simulink library "mssSimulink"  (R2024a)
settings: Solver=ode45  StartTime=0.0  StopTime=10.0  RelTol=1e-3
undefined symbols (not defined in the file): ABC, CN_data, CX_data, CY_data, D, G, Hoerner, K_supply, kt2ms, MA, magnitude, MRB, pathlength, RAO_Amp, RAO_Dir, RAO_Freq, RAO_Phase, RAO_Vel, RAO_yaw_back, RAO_yaw_quant, RAO_yaw_quantization_flag, rho_a, slcm, T_supply, table, vessel, vesselABC
libraries: $bdroot x99, simulink x13
(part 1 of 9)
settings Model: Creator=tristan  LastModifiedBy=thor
settings SolverCC: AlgebraicLoopSolver=TrustRegion
settings DataIOCC: LimitDataPoints=on  SaveFormat=Array  SignalLoggingSaveFormat=ModelDataLogs  ReturnWorkspaceOutputs=off
settings OptimizationCC: BlockReduction=off  BooleanDataType=off  ExpressionDepthLimit=2147483647  LifeSpan=inf
settings DebuggingCC: SaveWithParameterizedLinksMsg=none  UnderspecifiedInitializationDetection=Classic  MergeDetectMultiDrivingBlocksExec=none  SignalResolutionControl=TryResolveAllWithWarning  FcnCallInpInsideContextMsg=warning  UnconnectedInputMsg=warning  UnconnectedOutputMsg=warning  UnconnectedLineMsg=warning  StateNameClashWarn=warning  SFUnexpectedBacktrackingDiag=warning  SFNoUnconditionalDefaultTransitionDiag=warning  SFExecutionAtInitializationDiag=none  ArithmeticOperatorsInVariantConditions=warning
settings HardwareCC: ProdBitPerPointer=32  ProdBitPerSizeT=32  ProdBitPerPtrDiffT=32  ProdLargestAtomicFloat=None  ProdIntDivRoundTo=Undefined  ProdEndianess=Unspecified  ProdWordSize=32  ProdHWDeviceType=32-bit Generic  TargetUnknown=on
settings ModelReferenceCC: EnableRefExpFcnMdlSchedulingChecks=on  PropagateSignalLabelsOutOfModel=off
settings SFSimCC: SimUseLocalCustomCode=off  CustomCodeUndefinedFunction=UseInterfaceOnly
settings RTWCC: RTWUseLocalCustomCode=off  GPUComputeCapability=3.5  DLArmComputeVersion=19.05
settings CodeAppCC: StateflowObjectComments=on
settings GRTTargetCC: TargetLangStandard=C89/C90 (ANSI)  CombineOutputUpdateFcns=off  GRTInterface=on
settings ConfigComp: CovMetricSettings=dw  CovSaveCumulativeToWorkspaceVar=on  CovSaveSingleToWorkspaceVar=on  CovExternalEMLEnable=off

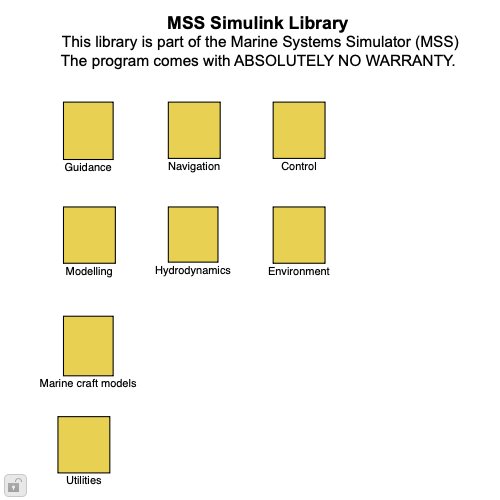
[thumbnail: Simulink's stored preview of the top-level diagram]
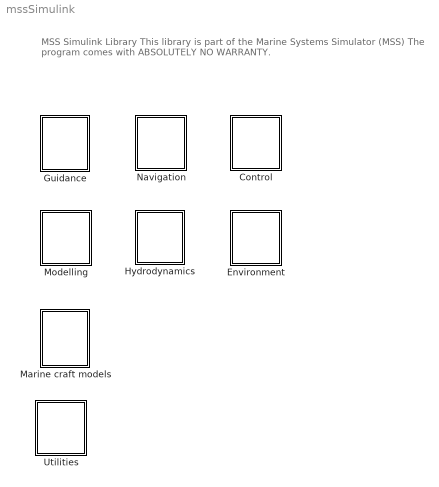
== system mssSimulink ==
  note: MSS Simulink Library
      | This library is part of the Marine Systems Simulator (MSS)
      | The program comes with ABSOLUTELY NO WARRANTY.
  Control : Subsystem
  Environment : Subsystem
  Guidance : Subsystem
  Hydrodynamics : Subsystem
  Marine craft models : Subsystem
  Modelling : Subsystem
  Navigation : Subsystem
  Utilities : Subsystem

== system mssSimulink/Control ==
  Autopilots : Subsystem
  DP : Subsystem

== system mssSimulink/Environment ==
  Current : Subsystem
  Waves : Subsystem
  Wind : Subsystem

== system mssSimulink/Guidance ==
  ALOS guidance law for heading autopilot : MATLAB Function  InitFcn=clear ILOSpsi  TreatAsAtomicUnit=on
  ILOS guidance law for heading autopilot : MATLAB Function  InitFcn=clear ILOSpsi  TreatAsAtomicUnit=on
  LOS guidance law for course autopilot : MATLAB Function  InitFcn=clear LOSchi  TreatAsAtomicUnit=on
  LOS observer : Subsystem  mask(LOS observer){K_f=0.3, alpha=5}
      mask prompts: K_f "Observer gain"; alpha "Bandwidth ratio between the differentiator and the observer, typically 5 to 10"
      mask help:
      | LOSobserver estimates the desired Line-Of-Sight (LOS) angle and rate from a LOS guidance law command, LOScommand[k]. The observer is
      |
      |   LOSangle[k+1] = LOSangle[k] + h * ( LOSrate[k] + K_f * ssa(LOScommand[k] - LOSangle[k]))
      |
      | where the LOS yaw rate is computed using numerical differentiation, LOSrate = T_f*s / (T_f*s + 1) * LOSangle. Exact discretization gives (Fossen 2021, Eqs. B.46-B.47)
      |
      |   LOSratek] = LOSangle[k][k] - xi[k]
      |   xi[k+1] = exp(-h/T_f) * xi[k] + (1 - exp(-h/T_f)) * LOSangle[k]
      |
      | where
      |
      |   K_f: Observer gain, LOSangle (typically 0.1-0.5)
      |   T_f:  Differentiator time constant,  LOSrate = T_f*s / (T_f*s + 1) * LOSangle
      |
      | Typically, the LOSrate loop is chosen 5 times faster than the LOSangle loop, that is 1/T_f = alpha * K_f where alpha = 5
      mask Display:
      | disp('Observer')
      | port_label('output', 2, 'LOSrate')
      | port_label('output', 1, 'LOSangle')
      | port_label('input', 1, 'LOScommand')
  Reference model : Subsystem  mask(3rd-order reference model){v_max=1.0, zeta_d=1.0, w_d=0.1}
      mask prompts: v_max "Max. velocity:"; zeta_d "Relative damping ratio:"; w_d "Natural frequency:"
      mask help: 3rd-order reference model with velocity saturation.
      mask Display:
      | disp('3rd order \nLP-filter')
      | port_label('output', 3, 'acc_d')
      | port_label('output', 2, 'vel_d')
      | port_label('output', 1, 'mag_d')
      | port_label('input', 1, 'ref')
  Waypoint guidance block : Subsystem  mask(Guidance){x_vector=[-800 -500 -200 -50 -200 -250 200 500 500 300 0 -300 -600], y_vector=[100 1800 2000 1500 1000 100 1000 300 -250 -200 100 -600 -1000], method=5th order polynomial, drawmode=off, stop=on, mode=Acc, start=[100 0], final=[0 100], constraint=off}
      mask prompts: x_vector "X value"; y_vector "Y value"; method "Computation method for path generation"; drawmode "Draw an extra plot showing the path with waypoints"; stop "Stop simulation when last waypoint is reached"; mode "Use constraints on acceleration or velocity in the endpoints"; start "Constraints in first waypoint [x, y]. (Only applicable for cubic splines)"; final "Constraints in last waypoint [x, y]. (Only applicable for cubic splines)"; constraint "Use constraints on the derivatives (Only applicable for 5th order)"
      mask help:
      | Way-Point Guidance Block
      | Author:  Jorgen Corneliussen
      | Date:     20 November 2002
      |
      | Creates a three times differentiable path between the waypoints provided. The user can choose between cubic splines and polinomial interpolation.
      |
      | NOTE: You have to supply the actual waypoints for the path generation.
      mask init:
      | if method == 1
      | 	[table, pathlength] = order3(x_vector,y_vector, drawmode, mode, start(1), final(1), start(2), final(2));
      | elseif method == 2
      | 	[table, pathlength] = order5(drawmode, constraint, x_vector, y_vector);
      | else
      | 	disp('Error in block initialization')
      | end
      mask Help:
      | <p>Way-Point Guidance Block<br>
      |   Author: Jorgen Corneliussen<br>
      |   Date: 20 November 2002</p>
      | <ul>
      |   <li> The input vectors must be of the same length, and contain the coordinates
      |     of the waypoints.</li>
      |   <li>If chosen, the block can draw an extra plot showing the path and the waypoints.</li>
      |   <li> The field &quot;Computation method&quot; allows the user to choose between
      |     a third and fifth order polynomal for path generation. </li>
      |   <li>If &quot;Stop simulation&quot; is not checked, the velocity input to the
      |     block is set to zero when the last waypoint is reached. </li>
      |   <li>For the third order algorithm, the user can choose between having endpoint
      |     constraints in velocity or acceleration. The values must be provided in the
      |     specified fields.</li>
      |   <li>For the fifth order polynomial, the user can choose to constrain the derivatives
      |     in the waypoints. This might in some cases reduce oscillations.<br>
      |   </li>
      | </ul>
      mask TypeOptions method: Cubic spline | 5th order polynomial
      mask TypeOptions mode: Vel | Acc
      mask Display:
      | image(imread('simulink/figs/compass.jpg'))
      | 
      | color('black'); port_label('output', 1, 'xy')
      | color('black'); port_label('output', 2, 'eta_vec')
      | color('black'); port_label('output', 3, 'vs_tot')
      | 
      | color('black'); port_label('input', 1, 'ud_total')
      | color('black'); port_label('input', 2, 'theta')
  "Zigzag test rudder command " : Subsystem  mask(Z- Manoeuvre test or Zig-Zag test){RL=[]}
      mask prompts: RL "Maximum rudder angle [rad]:"
      mask help:
      | This block generates the rudder command for a Z-manoeuvre test
      | IMO A601, ITTC 1975, SNAME 1989.
      | Copyright (C) 2005 NTNU
      |  Author: Tristan Perez

== system mssSimulink/Hydrodynamics ==
  6-DOF DP model (zero-speed model with fluid memory) : Subsystem  mask(6 DOF zero speed model){ABC=vesselABC, rho=1025, Axc=0.9*vessel.main.T*vessel.main.B, Ayc=0.9*vessel.main.T*vessel.main.Lpp, CX=1, CY_2D=Hoerner(vessel.main.B,vessel.main.T)}
      mask prompts: ABC "Structure containing model parameters and the fluid memory effects"; rho "Density of water (kg/m3)"; Axc "Frontal projected current area Axc (m2)"; Ayc "Laterall projected current area Ayc (m2)"; CX "Current (drag) coefficient in surge CX"; CY_2D "2D drag coefficient in sway CY_2D"
      mask help: System block containing the zero speed 6 DOF equations of motion including fluid memory effetcs.
  6-DOF maneuvering model (unified model with fluid memory) : Subsystem  mask(ShipX (Veres) 6 DOF unified DP and maneuvering model){ABC=vesselABC, rho=1025, Axc=0.9*vessel.main.T*vessel.main.B, Ayc=0.9*vessel.main.T*vessel.main.Lpp, CX=1, CY_2D=Hoerner(vessel.main.B,vessel.main.T)}
      mask prompts: ABC "Structure containing the fluid memory effects"; rho "Density of water (kg/m3)"; Axc "Frontal projected current area (m2)"; Ayc "Lateral projected current area (m2)"; CX "Current (drag) coefficient in surge CX"; CY_2D "2D drag coefficient in sway CY_2D"
      mask help:
      | System block containing the Shipx (Veres) 6 DOF unified DP and maneuvering model. The  6 DOF equations of motion also includes fluid memory effetcs. The data structure:
      |
      |    ABC.*           (>> load ABC )
      |
      | is generated using the Matlab script:
      |
      |    >> veres2ABC.m
      |
      | This script computes the retardation functions using state-space model approximations. It is also possible to include frequency-dependent viscous effects my editing the script.
      |
      | Author: Thor I. Fossen
      | -------------------------------------------------------------------------------------------------------------------------------------------------------
      | Reference:
      | T. I. Fossen and Ø. Smogeli (2004). Nonlinear Time-Domain Strip Theory Formulation for Low-Speed Maneuvering and Station-Keeping, Modelling, Identification and Control, MIC-25 (4):201-221.
      |
      | T. I. Fossen. A Nonlinear Unified State-Space Model for Ship Maneuvering and Control in a Seaway.  Journal of Bifurcation and Chaos (ENOC'05 Plenary), 2005.
  Cross-flow drag and surge resistance : Subsystem  TreatAsAtomicUnit=on  mask(Cross-flow drag and surge resistance){N=20, Lpp=vessel.main.Lpp, CD=0.5, Cx=0.5, Ax=100, Ay=500, rho_w=1025}
      mask prompts: N "Number of cross sections"; Lpp "Length between perpendiculars (m)"; CD "2D transversal drag coefficient CY  (-)"; Cx "3D drag coefficient in surge (-)"; Ax "Frontal current area Ax (m2)"; Ay "Transversal area (m2)"; rho_w "Density of water (kg/m^3)"
      mask help:
      | The viscous current loads in sway and yaw are computed using the cross-flow principle (pp. 187-197, Faltinsen 1990). 2-D drag coefficients CY_2D are used for each section of the hull. Integration over the length Lpp of the ship is performed using the trapezoidal rule. The forces are:
      |
      | Y = 0.5*rho_w*(Ay/Lpp)*CY_2D*Integral_{-0.5*Lpp}^{0.5*Lpp}  (v+x*r)|v+x*r| dx
      | N = 0.5*rho_w*(Ay/Lpp)*CY_2D*Integral_{-0.5*Lpp}^{0.5*Lpp}  x*(v+x*r)|v+x*r| dx
      |
      | where CY_2D is the 2D drag coefficient e.g. computed using Hoerner's formula.
      |
      | In surge the viscous resistance is modelled as quadratic drag:
      |
      | X = 0.5*rho_w*CX*Ax*u*|u|
      |
      | where Cx is the 3D drag coefficient in surge.
      |
      | Author: Thor I. Fossen
      mask init:
      | % ITTC drag
      | epsilon = 201; % ensure that log10(Rn)>2.0
      | 
      | Rn_min = 1e6;  % minimum Reynold's tall
      | %Ct_max = 0.075*(1+k)/(log10(Rn_min)-2)^2;
      | 
      | %S = Lpp*(B+2*T);
      mask Help:
      | <p>The viscous current loads in sway and yaw are computed using the cross-flow principle (pp. 187-197, Faltinsen 1990). 2-D drag coefficients CY_2D are used for each section of the hull. Integration over the length L of the ship is performed using the trapezoidal rule. The forces are:</p>
      | <p>Y = 0.5*rho_w*(Ay/Lpp)*CY_2D*Integral_{-0.5*Lpp}^{0.5*Lpp}  (v+x*r)|v+x*r| dx</p>
      | <p>N = 0.5*rho_w*(Ay/Lpp)*CY_2D*Integral_{-0.5*Lpp}^{0.5*Lpp}  x*(v+x*r)|v+x*r| dx</p>
      | where CY_2D is the 2D drag coefficient e.g. computed using Hoerner's formula.
      | <p>
      | In surge the viscous resistance is modelled as quadratic drag:
      | </p>
      | <p>
      | X = 0.5*rho_w*CX*Ax*u*|u|
      | </p>
      | <p>where Cx is the 3D drag coefficient in surge.<br>
      | </p>
      | <p>Author: Thor I. Fossen</p>
  Fluid memory effetcs : Subsystem
  Motion RAO (U=0) : Subsystem  mask(Motion RAO){RAO_Freq=vessel.motionRAO.w, RAO_Dir=vessel.headings, RAO_Vel=vessel.velocities, RAO_Amp=vessel.motionRAO.amp, RAO_Phase=vessel.motionRAO.phase, RAO_add_omega_0=on, RAO_add_omega_inf=on, RAO_yaw_quantization_flag=on, RAO_yaw_quant=5*pi/180, RAO_yaw_back=1.2*pi/180, RAO_speed_backlash_flag=on, RAO_speed_back=2, RAO_smoothing_flag=on}
      mask prompts: RAO_Freq "Vector of frequencies RAO_Freq (rad/s)"; RAO_Dir "Vector of directions RAO_Dir (rad)"; RAO_Vel "Vector of velocities RAO_Vel (m/s)"; RAO_Amp "6DOF Cell array with tables of Amplitudes RAO_Amp"; RAO_Phase "6DOF Cell array with tables of Phases RAO_Phase (rad)"; RAO_add_omega_0 "Add asymptotic RAO values for omega = 0"; RAO_add_omega_inf "Add asymptotic RAO values for omega = inf"; RAO_yaw_quantization_flag "LF estimator for yaw angle table lookup (backlash and quantization)"; RAO_yaw_quant "LF yaw angle quantization interval [rad]"; RAO_yaw_back "LF yaw angle backlash width [rad] (typically 1/4 of the quantization interval)"; RAO_speed_backlash_flag "Speed lookup backlash (avoid rapid speed data switching)"; RAO_speed_back "Speed backlash widht [m/s]"; RAO_smoothing_flag "Smooth the output to avoid switching transients due to table lookup"
      mask help:
      | Calculate the wave-frequency motion of a vessel in 6 degrees-of-freedom (DOF) from its Motion Response Amplitude Operators (Motion RAOs) and a sea state defined by a set of harmonic waves. The block takes the "Waves" bus from the MSS Waves block as input, as well as the vessel low-frequency (LF) motion in terms of the generalized position vector eta_LF and mean surge velocity U. See help for details.
      |
      | Copyright (C) NTNU 2005
      | Author: Oyvind N. Smogeli, 2005-05-03
      mask init:
      | % use only nonzero increasing velocities, if zero element add eps
      | Nvel = length(RAO_Vel);
      | 
      | if Nvel == 1
      |     RAO_Vel = [0 1e10];   % use one data set for U=0 and one dummy set for u=1e10
      |     Nvel = 2;
      | end
      | 
      | for dof = 1:6
      |     TempA{dof}  = RAO_Amp{dof}(:,:,1:Nvel);
      |     TempP{dof}  = RAO_Phase{dof}(:,:,1:Nvel);
      | end
      | 
      | clear RAO_Amp RAO_Phase
      | 
      | RAO_Amp   = TempA;
      | RAO_Phase = TempP;
      | 
      | % Add RAO values for zero frequency: use values for lowest given frequency
      | if RAO_add_omega_0 > 0
      | 	
      | 	if min(RAO_Freq) > 0
      | 				
      | 		RAO_Freq = [0 RAO_Freq];
      | 		
      | 		for dofno = 1:6
      | 			RAO_Amp{dofno} = [RAO_Amp{dofno}(1,:,:); RAO_Amp{dofno}];
      | 			RAO_Phase{dofno} = [RAO_Phase{dofno}(1,:,:); RAO_Phase{dofno}];
      | 		end
      | 	
      | 	end
      | 	
      | end
      | 
      | % Add RAO values for high frequency: use values for highest given frequency
      | maxfreq = 10;
      | if RAO_add_omega_inf > 0
      | 
      | 	if max(RAO_Freq) < maxfreq
      | 			
      | 		newfreq = 2*max(RAO_Freq) - RAO_Freq(length(RAO_Freq)-1);
      |         if newfreq > maxfreq
      |             newfreq = maxfreq - 0.1;
      |         end
      | 		
      | 		RAO_Freq = [RAO_Freq newfreq maxfreq];
      | 		
      | 		for dofno = 1:6
      | 			RAO_Amp{dofno} = [RAO_Amp{dofno} ; zeros(2, length(RAO_Dir), length(RAO_Vel))];
      | 			RAO_Phase{dofno} = [RAO_Phase{dofno} ; zeros(2, length(RAO_Dir), length(RAO_Vel))];
      | 		end
      | 		
      | 	end
      | 
      | end
      mask Help:
      | <b>Part of the Marine Systems Simulator: MSS</b><br>
      | <br>
      | Calculate the wave-frequency motion of a vessel in 6 degrees-of-freedom (DOF)
      | from its Motion Response Amplitude Operators (Motion RAOs) and a sea state
      | defined by a set of harmonic waves. The block takes the &quot;Waves&quot; bus from the MSS
      | Waves block as input, as well as the vessel low-frequency (LF) motion in terms
      | of the generalized position vector Eta_LF and surge velocity U.<p>
      | The Motion RAOs are defined in terms of a vector of frequencies (RAO_Freq), a
      | vector of directions (RAO_Dir), a vector of velocities (RAO_Dir), a 6DOF cell
      | array of 3D matrices with amplitudes (RAO_Amp), and a 6DOF cell array of 3D
      | matrices with phases (RAO_Phase), which are all input in the block mask. The
      | first dimension of the 3D matrices corresponds to the frequencies, the second to
      | the directions, and the third to the velocities, such that e.g. the amplitude
      | amp in heave (DOF #3) for frequency number n_f, direction number n_d and
      | velocity number n_v can be found from a = RAO_Amp{3}(n_f, n_d, n_v). </p>
      | <p><b>Inputs:</b></p>
      | <p>Waves:&nbsp;&nbsp;&nbsp;&nbsp;&nbsp;&nbsp;&nbsp;&nbsp;&nbsp;&nbsp;&nbsp; Bus
      | containing the following signals<br>
      | &nbsp;&nbsp;&nbsp; Zeta_a:&nbsp;&nbsp;&nbsp;&nbsp;&nbsp;&nbsp;&nbsp; Vector of harmonic wave amplitudes [m]<br>
      | &nbsp;&nbsp;&nbsp; Omega:&nbsp;&nbsp;&nbsp;&nbsp;&nbsp;&nbsp; Vector of harmonic wave frequencies [rad/s]<br>
      | &nbsp;&nbsp;&nbsp; Phase:&nbsp;&nbsp;&nbsp;&nbsp;&nbsp;&nbsp;&nbsp;&nbsp; Vector of harmonic wave phases (random) [rad]<br>
      | &nbsp;&nbsp;&nbsp; Wavenum:&nbsp;&nbsp;&nbsp; Vector of harmonic wave numbers [1/m]<br>
      | &nbsp;&nbsp;&nbsp; Psi:&nbsp;&nbsp;&nbsp;&nbsp;&nbsp;&nbsp;&nbsp;&nbsp;&nbsp;&nbsp;&nbsp;&nbsp;&nbsp; Vector of harmonic wave directions [rad]</p>
      | <p>eta_LF:&nbsp;&nbsp;&nbsp;&nbsp;&nbsp;&nbsp;&nbsp;&nbsp;&nbsp;&nbsp;&nbsp;
      | Generalized 6DOF n-frame low-frequency position vector [x (m), y (m), z (m),
      | theta (rad), phi (rad), psi (rad)]<br>
      | U:&nbsp;&nbsp;&nbsp;&nbsp;&nbsp;&nbsp;&nbsp;&nbsp;&nbsp;&nbsp;&nbsp;&nbsp;&nbsp;&nbsp;&nbsp;&nbsp;&nbsp;&nbsp;&nbsp;
      | Low-frequency (mean) surge velocity&nbsp; [m/s]</p>
      | <p><b>Outputs:</b></p>
      | <p>eta_WF:&nbsp;&nbsp;&nbsp;&nbsp;&nbsp;&nbsp;&nbsp;&nbsp;&nbsp; Generalized
      | 6DOF n-frame wave-frequency position vector [x (m), y (m), z (m), theta (rad),
      | phi (rad), psi (rad)]<br>
      | nu_WF:&nbsp;&nbsp;&nbsp;&nbsp;&nbsp;&nbsp;&nbsp;&nbsp;&nbsp;&nbsp; Generalized
      | 6DOF h-frame wave-frequency velocity vector [u (m/s), v (m/s), w (m/s), p
      | (rad/s), q (rad/s), r (rad/s)]<br>
      | nu_dot_WF:&nbsp;&nbsp;&nbsp;&nbsp; Generalized 6DOF h-frame wave-frequency
      | acceleration vector d/dt([u (m/s), v (m/s), w (m/s), p (rad/s), q (rad/s), r
      | (rad/s)])</p>
      | <p><b>Model validity:</b></p>
      | <p>The validity of the block is dependent on the validity of the given
      | RAO data set.</p>
      | <p>A proper RAO to be used with this block should contain at least 1 velocity, 5
      | directions (e.g. 0, 45, 90, 135 and 180 degrees) and 10-20 frequencies, for all
      | 6 DOF (surge, sway, heave, roll, pitch, yaw).</p>
      | <p>The block performs linear interpolation in frequencies and directions, and
      | uses the data set for the velocity closest to the input velocity (i.e. 'nearest'
      | interpolation in velocity). If the block recieves an input wave frequency or relative
      | wave direction outside the span of the data vectors RAO_Freq or RAO_Dir
      | respectively, the simulation stops and an error is returned. This means that a well-defined
      | RAO must contain data for both 0 and 180 degrees, and for frequencies covering
      | the desired range of wave frequencies. If desired, asymptotic values can be
      | automatically added for zero and infinity frequency to avoid runtime errors if
      | the wave freqeuncy exceeds the values in RAO_Freq (see checkboxes in the mask). </p>
      | <p>IMPORTANT NOTE: The RAO theory upon which this block is based is in reality
      | only valid when the vessel low-frequency (h-frame) motion is a constant surge
      | velocity only, and the vessel is performing wave-frequency oscillations about
      | the steadily translating h-frame.This means that the outputs from the block when
      | manoeuvering -- i.e. changing the surge velocity and/or yaw angle -- must be
      | interpreted with some care. A jump in the output must be expected when changing
      | between two velocity data sets, and frequency warping expected when changing the
      | yaw angle (due to interpolation in the phase). It is therefore recommended to
      | use backlash on the input velocity to avoid transient switching, and a quantized
      | yaw angle with backlash. The latter will lead to jump in the ouput when the yaw
      | angle changes from one quantizied value to another, but will give better results
      | when keeping within one quantizer interval. The quantized yaw angle with
      | backlash and velocity with backlash are available as options via checkboxes in
      | the mask. If either of these are activated, proper values for the yaw
      | quantization interval, yaw backlash width, and the the speed backlash width
      | respectively must be set. Typical values could be a yaw quantization interval of
      | 5 degrees, yaw backlash width of 1/4-1/5 of the quantization interval, and speed
      | backlash width of 1 m/s. To avoid the most rapid transients when switching
      | between data sets, output smoothing is available as an option in the mask. If
      | this is enabled, the output during a transent is rate limited according to the
      | fastest recorded signal rate during normal operation.</p>
      | <p><b>Example mask input:</b></p><p>
      | As an example, the format of the mask input for 2 velocities, 3 directions and 5
      | frequencies is as follows:<p>RAO_Freq = [f1 f2 f3 f4 f5]<br>
      | RAO_Dir = [d1 d2 d3]<br>
      | RAO_Vel = [v1 v2]<p>Surge:<br>
      | RAO_Amp{1}(:,:,1)&nbsp; = [a1_111 a1_121 a1_131; a1_211 a1_221 a1_231; a1_311
      | a1_321 a1_331; a1_411 a1_421 a1_431; a1_511 a1_521 a1_531]<br>
      | RAO_Amp{1}(:,:,2)&nbsp; = [a1_112 a1_122 a1_132; a1_212 a1_222 a1_232; a1_312
      | a1_322 a1_332; a1_412 a1_422 a1_432; a1_512 a1_522 a1_532]<br>
      | RAO_Phase{1}(:,:,1) = [p1_111 p1_121 p1_131; p1_211 p1_221 p1_231; p1_311 p1_321
      | p1_331; p1_411 p1_421 p1_431; p1_511 p1_521 p1_531]<br>
      | RAO_Phase{1}(:,:,2) = [p1_112 p1_122 p1_132; p1_212 p1_222 p1_232; p1_312 p1_322
      | p1_332; p1_412 p1_422 p1_432; p1_512 p1_522 p1_532]<p>Sway:<br>
      | RAO_Amp{2}(:,:,1)&nbsp; = [a2_111 a2_121 a2_131; a2_211 a2_221 a2_231; a2_311
      | a2_321 a2_331; a2_411 a2_421 a2_431; a2_511 a2_521 a2_531]<br>
      | RAO_Amp{2}(:,:,2)&nbsp; = [a2_112 a2_122 a2_132; a2_212 a2_222 a2_232; a2_312
      | a2_322 a2_332; a2_412 a2_422 a2_432; a2_512 a2_522 a2_532]<br>
      | RAO_Phase{2}(:,:,1) = [p2_111 p2_121 p2_131; p2_211 p2_221 p2_231; p2_311 p2_321
      | p2_331; p2_411 p2_421 p2_431; p2_511 p2_521 p2_531]<br>
      | RAO_Phase{2}(:,:,2) = [p2_112 p2_122 p2_132; p2_212 p2_222 p2_232; p2_312 p2_322
      | p2_332; p2_412 p2_422 p2_432; p2_512 p2_522 p2_532]<p>....<p>Yaw:<br>
      | RAO_Amp{6}(:,:,1)&nbsp; = [a6_111 a6_121 a6_131; a6_211 a6_221 a6_231; a6_311
      | a6_321 a6_331; a6_411 a6_421 a6_431; a6_511 a6_521 a6_531]<br>
      | RAO_Amp{6}(:,:,2)&nbsp; = [a6_112 a6_122 a6_132; a6_212 a6_222 a6_232; a6_312
      | a6_322 a6_332; a6_412 a6_422 a6_432; a6_512 a6_522 a6_532]<br>
      | RAO_Phase{6}(:,:,1) = [p6_111 p6_121 p6_131; p6_211 p6_221 p6_231; p6_311 p6_321
      | p6_331; p6_411 p6_421 p6_431; p6_511 p6_521 p6_531]<br>
      | RAO_Phase{6}(:,:,2) = [p6_112 p6_122 p6_132; p6_212 p6_222 p6_232; p6_312 p6_322
      | p6_332; p6_412 p6_422 p6_432; p6_512 p6_522 p6_532]<p>where now for example the
      | amplitude and phase in sway (DOF 2) for frequency f5, direction d3 and velocity
      | v1 are given by RAO_Amp{2}(5,3,1) = a2_531 and RAO_Phase{2}(5,3,1) = p2_531.<p>
      | <b>Copyright (C) NTNU 2005</b></p>
      | <p><b>Author:</b> Oyvind N. Smogeli, 2005-05-03</p></body>
  WD for heading1 : Subsystem  mask(Force RAO){ForceRAO_Freq=vessel.forceRAO.w, WD_Freq=vessel.driftfrc.w, RAO_Vel=vessel.velocities, ForceRAO_Amp=vessel.forceRAO.amp, ForceRAO_Phase=vessel.forceRAO.phase, WD_Amp=vessel.driftfrc.amp, RAO_add_omega_0=on, RAO_add_omega_inf=on}
      mask prompts: ForceRAO_Freq "Vector of frequencies ForceRAO_Freq (rad/s)"; WD_Freq "Vector of frequencies WD_Freq (rad/s)"; RAO_Vel "Vector of velocities RAO_Vel (m/s)"; ForceRAO_Amp "6DOF Cell array with tables of Amplitudes ForceRAO_Amp"; ForceRAO_Phase "6DOF Cell array with tables of Phases ForceRAO_Phase (rad)"; WD_Amp "6DOF Cell array with tables of Amplitudes WD_Amp"; RAO_add_omega_0 "Add asymptotic RAO values for omega = 0"; RAO_add_omega_inf "Add asymptotic RAO values for omega = inf"
      mask help:
      | Calculate the 6 degrees-of-freedom (DOF) wave-frequency excitation forces tau_WF for a vessel from its Force Response Amplitude Operators (Force RAOs) and a sea state defined by a set of harmonic waves. The block takes the "Waves" bus from the MSS Waves block as input, as well as the vessel low-frequency (LF) motion in terms of the generalized position vector eta and mean surge velocity U. See help for details.
      |
      | Authors: Oyvind N. Smogeli and Thor I. Fossen, 2005-05-03
      mask init:
      | % use only nonzero increasing velocities, if zero element add eps
      | Nvel = length(RAO_Vel);
      | 
      | if Nvel == 1
      |     RAO_Vel = [0 1e10];   % use one data set for U=0 and one dummy set for u=1e10
      |     Nvel = 2;
      | end
      | 
      | for dof = 1:3
      |     TempWA{dof}  = WD_Amp{dof}(:,:,1:Nvel);
      | end
      | 
      | clear WD_Amp WD_Phase
      | 
      | WD_Amp         = TempWA;
      | 
      | % Add RAO values for zero frequency: use values for lowest given frequency
      | if RAO_add_omega_0 > 0
      | 	 
      | 	if min(WD_Freq) > 0
      |         
      | 		WD_Freq = [0 WD_Freq];
      | 		for dofno = 1:3
      | 			WD_Amp{dofno} = [WD_Amp{dofno}(1,:,:); WD_Amp{dofno}];
      | 		end        
      |         
      | 	end
      | 	
      | end
      | 
      | % Add RAO values for high frequency: use values for highest given frequency
      | maxfreq = 10;
      | if RAO_add_omega_inf > 0
      | 
      | 	if max(WD_Freq) < maxfreq
      | 			
      | 		newfreq = max(WD_Freq) + 0.5*(maxfreq-max(WD_Freq));
      |         
      | 		WD_Freq = [WD_Freq newfreq maxfreq];
      | 		for dofno = 1:3
      | 			WD_Amp{dofno} = [WD_Amp{dofno}; zeros(2, 36, Nvel)];
      | 		end
      | 		
      |     end
      |     
      | end
      mask Help:
      | <b>Part of the Marine Systems Simulator: MSS</b><br>
      | <br>
      | Calculate the 6 degrees-of-freedom (DOF) wave-frequency excitation forces tau_WF
      | for a vessel from its Force Response Amplitude Operators (Force RAOs) and a sea
      | state defined by a set of harmonic waves. The block takes the &quot;Waves&quot; bus from
      | the MSS Waves block as input, as well as the vessel low-frequency (LF) motion in
      | terms of the generalized position vector eta and mean surge velocity U.<p>The Force RAOs are defined in terms of a
      | vector of frequencies (RAO_Freq), a vector of directions (RAO_Dir), a vector of
      | velocities (RAO_Dir), a 6DOF cell array of 3D matrices with amplitudes
      | (RAO_Amp), and a 6DOF cell array of 3D matrices with phases (RAO_Phase), which
      | are all input in the block mask. The first dimension of the 3D matrices
      | corresponds to the frequencies, the second to the directions, and the third to
      | the velocities, such that e.g. the amplitude amp in heave (DOF #3) for frequency
      | number n_f, direction number n_d and velocity number n_v can be found from a =
      | RAO_Amp{3}(n_f, n_d, n_v).</p>
      | <p><b>Inputs:</b></p>
      | <p>Waves:&nbsp;&nbsp;&nbsp;&nbsp;&nbsp;&nbsp;&nbsp;&nbsp;&nbsp;&nbsp;&nbsp; Bus
      | containing the following signals<br>
      | &nbsp;&nbsp;&nbsp; Zeta_a:&nbsp;&nbsp;&nbsp;&nbsp;&nbsp;&nbsp;&nbsp; Vector of harmonic wave amplitudes [m]<br>
      | &nbsp;&nbsp;&nbsp; Omega:&nbsp;&nbsp;&nbsp;&nbsp;&nbsp;&nbsp; Vector of harmonic wave frequencies [rad/s]<br>
      | &nbsp;&nbsp;&nbsp; Phase:&nbsp;&nbsp;&nbsp;&nbsp;&nbsp;&nbsp;&nbsp;&nbsp; Vector of harmonic wave phases (random) [rad]<br>
      | &nbsp;&nbsp;&nbsp; Wavenum:&nbsp;&nbsp;&nbsp; Vector of harmonic wave numbers [1/m]<br>
      | &nbsp;&nbsp;&nbsp; Psi:&nbsp;&nbsp;&nbsp;&nbsp;&nbsp;&nbsp;&nbsp;&nbsp;&nbsp;&nbsp;&nbsp;&nbsp;&nbsp; Vector of harmonic wave directions [rad]</p>
      | <p>eta_LF:&nbsp;&nbsp;&nbsp;&nbsp;&nbsp;&nbsp;&nbsp;&nbsp;&nbsp;&nbsp;&nbsp;
      | Generalized 6DOF n-frame low-frequency position vector [x (m), y (m), z (m),
      | theta (rad), phi (rad), psi (rad)]<br>
      | U:&nbsp;&nbsp;&nbsp;&nbsp;&nbsp;&nbsp;&nbsp;&nbsp;&nbsp;&nbsp;&nbsp;&nbsp;&nbsp;&nbsp;&nbsp;&nbsp;&nbsp;&nbsp;&nbsp;
      | Low-frequency (mean) surge velocity&nbsp; [m/s]</p>
      | <p><b>Outputs:</b></p>
      | <p>tau_WF:&nbsp;&nbsp;&nbsp;&nbsp;&nbsp;&nbsp;&nbsp;&nbsp;&nbsp; Generalized
      | 6DOF h-frame force vector [X (N), Y (N), Z (N), K (Nm), M (Nm), N (Nm)]</p>
      | <p><b>Model validity:</b></p>
      | <p>The validity of the block is dependent on the validity of the given
      | RAO data set.</p>
      | <p>A proper RAO to be used with this block should contain at least 1 velocity, 5
      | directions (e.g. 0, 45, 90, 135 and 180 degrees) and 10-20 frequencies, for all
      | 6 DOF (surge, sway, heave, roll, pitch, yaw).</p>
      | <p>The block performs linear interpolation in frequencies and directions, and
      | uses the data set for the velocity closest to the input velocity (i.e. 'nearest'
      | interpolation in velocity). If the block recieves an input wave frequency or relative
      | wave direction outside the span of the data vectors RAO_Freq or RAO_Dir
      | respectively, the simulation stops and an error is returned. This means that a well-defined
      | RAO must contain data for both 0 and 180 degrees, and for frequencies covering
      | the desired range of wave frequencies. If desired, asymptotic values can be
      | automatically added for zero and infinity frequency to avoid runtime errors if
      | the wave freqeuncy exceeds the values in RAO_Freq (see checkboxes in the mask). </p>
      | <p>IMPORTANT NOTE: The RAO theory upon which this block is based is in reality
      | only valid when the vessel low-frequency (h-frame) motion is a constant surge
      | velocity only, and the vessel is performing wave-frequency oscillations about
      | the steadily translating h-frame.This means that the outputs from the block when
      | manoeuvering -- i.e. changing the surge velocity and/or yaw angle -- must be
      | interpreted with some care. A jump in the output must be expected when changing
      | between two velocity data sets, and frequency warping expected when changing the
      | yaw angle (due to interpolation in the phase). It is therefore recommended to
      | use backlash on the input velocity to avoid transient switching, and a quantized
      | yaw angle with backlash. The latter will lead to jump in the ouput when the yaw
      | angle changes from one quantized value to another, but will give better results
      | when keeping within one quantizer interval. The quantized yaw angle with
      | backlash and velocity with backlash are available as options via checkboxes in
      | the mask. If either of these are activated, proper values for the yaw
      | quantization interval, yaw backlash width, and the the speed backlash width
      | respectively must be set. Typical values could be a yaw quantization interval of
      | 5 degrees, yaw backlash width of 1/4-1/5 of the quantization interval, and speed
      | backlash width of 1 m/s. To avoid the most rapid transients when switching
      | between data sets, output smoothing is available as an option in the mask. If
      | this is enabled, the output during a transent is rate limited according to the
      | fastest recorded signal rate during normal operation.</p>
      | <p><b>Example mask input:</b></p><p>
      | As an example, the format of the mask input for 2 velocities, 3 directions and 5
      | frequencies is as follows:<p>RAO_Freq = [f1 f2 f3 f4 f5]<br>
      | RAO_Dir = [d1 d2 d3]<br>
      | RAO_Vel = [v1 v2]<p>Surge:<br>
      | RAO_Amp{1}(:,:,1)&nbsp; = [a1_111 a1_121 a1_131; a1_211 a1_221 a1_231; a1_311
      | a1_321 a1_331; a1_411 a1_421 a1_431; a1_511 a1_521 a1_531]<br>
      | RAO_Amp{1}(:,:,2)&nbsp; = [a1_112 a1_122 a1_132; a1_212 a1_222 a1_232; a1_312
      | a1_322 a1_332; a1_412 a1_422 a1_432; a1_512 a1_522 a1_532]<br>
      | RAO_Phase{1}(:,:,1) = [p1_111 p1_121 p1_131; p1_211 p1_221 p1_231; p1_311 p1_321
      | p1_331; p1_411 p1_421 p1_431; p1_511 p1_521 p1_531]<br>
      | RAO_Phase{1}(:,:,2) = [p1_112 p1_122 p1_132; p1_212 p1_222 p1_232; p1_312 p1_322
      | p1_332; p1_412 p1_422 p1_432; p1_512 p1_522 p1_532]<p>Sway:<br>
      | RAO_Amp{2}(:,:,1)&nbsp; = [a2_111 a2_121 a2_131; a2_211 a2_221 a2_231; a2_311
      | a2_321 a2_331; a2_411 a2_421 a2_431; a2_511 a2_521 a2_531]<br>
      | RAO_Amp{2}(:,:,2)&nbsp; = [a2_112 a2_122 a2_132; a2_212 a2_222 a2_232; a2_312
      | a2_322 a2_332; a2_412 a2_422 a2_432; a2_512 a2_522 a2_532]<br>
      | RAO_Phase{2}(:,:,1) = [p2_111 p2_121 p2_131; p2_211 p2_221 p2_231; p2_311 p2_321
      | p2_331; p2_411 p2_421 p2_431; p2_511 p2_521 p2_531]<br>
      | RAO_Phase{2}(:,:,2) = [p2_112 p2_122 p2_132; p2_212 p2_222 p2_232; p2_312 p2_322
      | p2_332; p2_412 p2_422 p2_432; p2_512 p2_522 p2_532]<p>...<p>Yaw:<br>
      | RAO_Amp{6}(:,:,1)&nbsp; = [a6_111 a6_121 a6_131; a6_211 a6_221 a6_231; a6_311
      | a6_321 a6_331; a6_411 a6_421 a6_431; a6_511 a6_521 a6_531]<br>
      | RAO_Amp{6}(:,:,2)&nbsp; = [a6_112 a6_122 a6_132; a6_212 a6_222 a6_232; a6_312
      | a6_322 a6_332; a6_412 a6_422 a6_432; a6_512 a6_522 a6_532]<br>
      | RAO_Phase{6}(:,:,1) = [p6_111 p6_121 p6_131; p6_211 p6_221 p6_231; p6_311 p6_321
      | p6_331; p6_411 p6_421 p6_431; p6_511 p6_521 p6_531]<br>
      | RAO_Phase{6}(:,:,2) = [p6_112 p6_122 p6_132; p6_212 p6_222 p6_232; p6_312 p6_322
      | p6_332; p6_412 p6_422 p6_432; p6_512 p6_522 p6_532]<p>where now for example the
      | amplitude and phase in sway (DOF 2) for frequency f5, direction d3 and velocity
      | v1 are given by RAO_Amp{2}(5,3,1) = a2_531 and RAO_Phase{2}(5,3,1) = p2_531.<p>
      | <b>Copyright (C) NTNU 2005</b></p>
      | <p><b>Author:</b> Oyvind N. Smogeli, 2005-05-03</p>
  Wave drift (U=0) : Subsystem
  Wave loads (U=0) : Subsystem
  Wave loads (U>0) : Subsystem
  Wave loads for heading1 : Subsystem  mask(Force RAO){ForceRAO_Freq=vessel.forceRAO.w, WD_Freq=vessel.driftfrc.w, RAO_Vel=vessel.velocities, ForceRAO_Amp=vessel.forceRAO.amp, ForceRAO_Phase=vessel.forceRAO.phase, WD_Amp=vessel.driftfrc.amp, RAO_add_omega_0=on, RAO_add_omega_inf=on}
      mask prompts: ForceRAO_Freq "Vector of frequencies ForceRAO_Freq (rad/s)"; WD_Freq "Vector of frequencies WD_Freq (rad/s)"; RAO_Vel "Vector of velocities RAO_Vel (m/s)"; ForceRAO_Amp "6DOF Cell array with tables of Amplitudes ForceRAO_Amp"; ForceRAO_Phase "6DOF Cell array with tables of Phases ForceRAO_Phase (rad)"; WD_Amp "6DOF Cell array with tables of Amplitudes WD_Amp"; RAO_add_omega_0 "Add asymptotic RAO values for omega = 0"; RAO_add_omega_inf "Add asymptotic RAO values for omega = inf"
      mask help:
      | Calculate the 6 degrees-of-freedom (DOF) wave-frequency excitation forces tau_WF for a vessel from its Force Response Amplitude Operators (Force RAOs) and a sea state defined by a set of harmonic waves. The block takes the "Waves" bus from the MSS Waves block as input, as well as the vessel low-frequency (LF) motion in terms of the generalized position vector eta and mean surge velocity U. See help for details.
      |
      | Authors: Oyvind N. Smogeli and Thor I. Fossen, 2005-05-03
      mask init:
      | % use only nonzero increasing velocities, if zero element add eps
      | Nvel = length(RAO_Vel);
      | 
      | if Nvel == 1
      |     RAO_Vel = [0 1e10];   % use one data set for U=0 and one dummy set for u=1e10
      |     Nvel = 2;
      | end
      | 
      | for dof = 1:6
      |     TempFA{dof}  = ForceRAO_Amp{dof}(:,:,1:Nvel);
      |     TempFP{dof}  = ForceRAO_Phase{dof}(:,:,1:Nvel);
      | end
      | 
      | for dof = 1:3
      |     TempWA{dof}  = WD_Amp{dof}(:,:,1:Nvel);
      | end
      | 
      | clear ForceRAO_Amp ForceRAO_Phase WD_Amp WD_Phase
      | 
      | ForceRAO_Amp   = TempFA;
      | ForceRAO_Phase = TempFP;
      | WD_Amp         = TempWA;
      | 
      | % Add RAO values for zero frequency: use values for lowest given frequency
      | if RAO_add_omega_0 > 0
      | 	
      | 	if min(ForceRAO_Freq) > 0
      | 				
      | 		ForceRAO_Freq = [0 ForceRAO_Freq];
      | 		for dofno = 1:6
      | 			ForceRAO_Amp{dofno}   = [ForceRAO_Amp{dofno}(1,:,:);   ForceRAO_Amp{dofno}];
      | 			ForceRAO_Phase{dofno} = [ForceRAO_Phase{dofno}(1,:,:); ForceRAO_Phase{dofno}];
      |         end
      | 
      |     end
      |     
      | 	if min(WD_Freq) > 0
      |         
      | 		WD_Freq = [0 WD_Freq];
      | 		for dofno = 1:3
      | 			WD_Amp{dofno} = [WD_Amp{dofno}(1,:,:); WD_Amp{dofno}];
      | 		end        
      |         
      | 	end
      | 	
      | end
      | 
      | % Add RAO values for high frequency: use values for highest given frequency
      | maxfreq = 10;
      | if RAO_add_omega_inf > 0
      | 
      | 	if max(ForceRAO_Freq) < maxfreq
      | 			
      | 		%newfreq = 2*max(ForceRAO_Freq) - ForceRAO_Freq(length(ForceRAO_Freq)-1);
      | 		newfreq = max(ForceRAO_Freq) + 0.5*(maxfreq-max(ForceRAO_Freq));
      |         
      | 		ForceRAO_Freq = [ForceRAO_Freq newfreq maxfreq];
      | 		for dofno = 1:6
      | 			ForceRAO_Amp{dofno}   = [ForceRAO_Amp{dofno};   zeros(2, 36, Nvel)];
      | 			ForceRAO_Phase{dofno} = [ForceRAO_Phase{dofno}; zeros(2, 36, Nvel)];
      | 		end
      | 		
      |     end
      | 
      | 	if max(WD_Freq) < maxfreq
      | 			
      | 		%newfreq = 2*max(WD_Freq) - WD_Freq(length(WD_Freq)-1);
      | 		newfreq = max(WD_Freq) + 0.5*(maxfreq-max(WD_Freq));
      |         
      | 		WD_Freq = [WD_Freq newfreq maxfreq];
      | 		for dofno = 1:3
      | 			WD_Amp{dofno} = [WD_Amp{dofno}; zeros(2, 36, Nvel)];
      | 		end
      | 		
      |     end
      |     
      | end
      mask Help:
      | <b>Part of the Marine Systems Simulator: MSS</b><br>
      | <br>
      | Calculate the 6 degrees-of-freedom (DOF) wave-frequency excitation forces tau_WF
      | for a vessel from its Force Response Amplitude Operators (Force RAOs) and a sea
      | state defined by a set of harmonic waves. The block takes the &quot;Waves&quot; bus from
      | the MSS Waves block as input, as well as the vessel low-frequency (LF) motion in
      | terms of the generalized position vector eta and mean surge velocity U.<p>The Force RAOs are defined in terms of a
      | vector of frequencies (RAO_Freq), a vector of directions (RAO_Dir), a vector of
      | velocities (RAO_Dir), a 6DOF cell array of 3D matrices with amplitudes
      | (RAO_Amp), and a 6DOF cell array of 3D matrices with phases (RAO_Phase), which
      | are all input in the block mask. The first dimension of the 3D matrices
      | corresponds to the frequencies, the second to the directions, and the third to
      | the velocities, such that e.g. the amplitude amp in heave (DOF #3) for frequency
      | number n_f, direction number n_d and velocity number n_v can be found from a =
      | RAO_Amp{3}(n_f, n_d, n_v).</p>
      | <p><b>Inputs:</b></p>
      | <p>Waves:&nbsp;&nbsp;&nbsp;&nbsp;&nbsp;&nbsp;&nbsp;&nbsp;&nbsp;&nbsp;&nbsp; Bus
      | containing the following signals<br>
      | &nbsp;&nbsp;&nbsp; Zeta_a:&nbsp;&nbsp;&nbsp;&nbsp;&nbsp;&nbsp;&nbsp; Vector of harmonic wave amplitudes [m]<br>
      | &nbsp;&nbsp;&nbsp; Omega:&nbsp;&nbsp;&nbsp;&nbsp;&nbsp;&nbsp; Vector of harmonic wave frequencies [rad/s]<br>
      | &nbsp;&nbsp;&nbsp; Phase:&nbsp;&nbsp;&nbsp;&nbsp;&nbsp;&nbsp;&nbsp;&nbsp; Vector of harmonic wave phases (random) [rad]<br>
      | &nbsp;&nbsp;&nbsp; Wavenum:&nbsp;&nbsp;&nbsp; Vector of harmonic wave numbers [1/m]<br>
      | &nbsp;&nbsp;&nbsp; Psi:&nbsp;&nbsp;&nbsp;&nbsp;&nbsp;&nbsp;&nbsp;&nbsp;&nbsp;&nbsp;&nbsp;&nbsp;&nbsp; Vector of harmonic wave directions [rad]</p>
      | <p>eta_LF:&nbsp;&nbsp;&nbsp;&nbsp;&nbsp;&nbsp;&nbsp;&nbsp;&nbsp;&nbsp;&nbsp;
      | Generalized 6DOF n-frame low-frequency position vector [x (m), y (m), z (m),
      | theta (rad), phi (rad), psi (rad)]<br>
      | U:&nbsp;&nbsp;&nbsp;&nbsp;&nbsp;&nbsp;&nbsp;&nbsp;&nbsp;&nbsp;&nbsp;&nbsp;&nbsp;&nbsp;&nbsp;&nbsp;&nbsp;&nbsp;&nbsp;
      | Low-frequency (mean) surge velocity&nbsp; [m/s]</p>
      | <p><b>Outputs:</b></p>
      | <p>tau_WF:&nbsp;&nbsp;&nbsp;&nbsp;&nbsp;&nbsp;&nbsp;&nbsp;&nbsp; Generalized
      | 6DOF h-frame force vector [X (N), Y (N), Z (N), K (Nm), M (Nm), N (Nm)]</p>
      | <p><b>Model validity:</b></p>
      | <p>The validity of the block is dependent on the validity of the given
      | RAO data set.</p>
      | <p>A proper RAO to be used with this block should contain at least 1 velocity, 5
      | directions (e.g. 0, 45, 90, 135 and 180 degrees) and 10-20 frequencies, for all
      | 6 DOF (surge, sway, heave, roll, pitch, yaw).</p>
      | <p>The block performs linear interpolation in frequencies and directions, and
      | uses the data set for the velocity closest to the input velocity (i.e. 'nearest'
      | interpolation in velocity). If the block recieves an input wave frequency or relative
      | wave direction outside the span of the data vectors RAO_Freq or RAO_Dir
      | respectively, the simulation stops and an error is returned. This means that a well-defined
      | RAO must contain data for both 0 and 180 degrees, and for frequencies covering
      | the desired range of wave frequencies. If desired, asymptotic values can be
      | automatically added for zero and infinity frequency to avoid runtime errors if
      | the wave freqeuncy exceeds the values in RAO_Freq (see checkboxes in the mask). </p>
      | <p>IMPORTANT NOTE: The RAO theory upon which this block is based is in reality
      | only valid when the vessel low-frequency (h-frame) motion is a constant surge
      | velocity only, and the vessel is performing wave-frequency oscillations about
      | the steadily translating h-frame.This means that the outputs from the block when
      | manoeuvering -- i.e. changing the surge velocity and/or yaw angle -- must be
      | interpreted with some care. A jump in the output must be expected when changing
      | between two velocity data sets, and frequency warping expected when changing the
      | yaw angle (due to interpolation in the phase). It is therefore recommended to
      | use backlash on the input velocity to avoid transient switching, and a quantized
      | yaw angle with backlash. The latter will lead to jump in the ouput when the yaw
      | angle changes from one quantized value to another, but will give better results
      | when keeping within one quantizer interval. The quantized yaw angle with
      | backlash and velocity with backlash are available as options via checkboxes in
      | the mask. If either of these are activated, proper values for the yaw
      | quantization interval, yaw backlash width, and the the speed backlash width
      | respectively must be set. Typical values could be a yaw quantization interval of
      | 5 degrees, yaw backlash width of 1/4-1/5 of the quantization interval, and speed
      | backlash width of 1 m/s. To avoid the most rapid transients when switching
      | between data sets, output smoothing is available as an option in the mask. If
      | this is enabled, the output during a transent is rate limited according to the
      | fastest recorded signal rate during normal operation.</p>
      | <p><b>Example mask input:</b></p><p>
      | As an example, the format of the mask input for 2 velocities, 3 directions and 5
      | frequencies is as follows:<p>RAO_Freq = [f1 f2 f3 f4 f5]<br>
      | RAO_Dir = [d1 d2 d3]<br>
      | RAO_Vel = [v1 v2]<p>Surge:<br>
      | RAO_Amp{1}(:,:,1)&nbsp; = [a1_111 a1_121 a1_131; a1_211 a1_221 a1_231; a1_311
      | a1_321 a1_331; a1_411 a1_421 a1_431; a1_511 a1_521 a1_531]<br>
      | RAO_Amp{1}(:,:,2)&nbsp; = [a1_112 a1_122 a1_132; a1_212 a1_222 a1_232; a1_312
      | a1_322 a1_332; a1_412 a1_422 a1_432; a1_512 a1_522 a1_532]<br>
      | RAO_Phase{1}(:,:,1) = [p1_111 p1_121 p1_131; p1_211 p1_221 p1_231; p1_311 p1_321
      | p1_331; p1_411 p1_421 p1_431; p1_511 p1_521 p1_531]<br>
      | RAO_Phase{1}(:,:,2) = [p1_112 p1_122 p1_132; p1_212 p1_222 p1_232; p1_312 p1_322
      | p1_332; p1_412 p1_422 p1_432; p1_512 p1_522 p1_532]<p>Sway:<br>
      | RAO_Amp{2}(:,:,1)&nbsp; = [a2_111 a2_121 a2_131; a2_211 a2_221 a2_231; a2_311
      | a2_321 a2_331; a2_411 a2_421 a2_431; a2_511 a2_521 a2_531]<br>
      | RAO_Amp{2}(:,:,2)&nbsp; = [a2_112 a2_122 a2_132; a2_212 a2_222 a2_232; a2_312
      | a2_322 a2_332; a2_412 a2_422 a2_432; a2_512 a2_522 a2_532]<br>
      | RAO_Phase{2}(:,:,1) = [p2_111 p2_121 p2_131; p2_211 p2_221 p2_231; p2_311 p2_321
      | p2_331; p2_411 p2_421 p2_431; p2_511 p2_521 p2_531]<br>
      | RAO_Phase{2}(:,:,2) = [p2_112 p2_122 p2_132; p2_212 p2_222 p2_232; p2_312 p2_322
      | p2_332; p2_412 p2_422 p2_432; p2_512 p2_522 p2_532]<p>...<p>Yaw:<br>
      | RAO_Amp{6}(:,:,1)&nbsp; = [a6_111 a6_121 a6_131; a6_211 a6_221 a6_231; a6_311
      | a6_321 a6_331; a6_411 a6_421 a6_431; a6_511 a6_521 a6_531]<br>
      | RAO_Amp{6}(:,:,2)&nbsp; = [a6_112 a6_122 a6_132; a6_212 a6_222 a6_232; a6_312
      | a6_322 a6_332; a6_412 a6_422 a6_432; a6_512 a6_522 a6_532]<br>
      | RAO_Phase{6}(:,:,1) = [p6_111 p6_121 p6_131; p6_211 p6_221 p6_231; p6_311 p6_321
      | p6_331; p6_411 p6_421 p6_431; p6_511 p6_521 p6_531]<br>
      | RAO_Phase{6}(:,:,2) = [p6_112 p6_122 p6_132; p6_212 p6_222 p6_232; p6_312 p6_322
      | p6_332; p6_412 p6_422 p6_432; p6_512 p6_522 p6_532]<p>where now for example the
      | amplitude and phase in sway (DOF 2) for frequency f5, direction d3 and velocity
      | v1 are given by RAO_Amp{2}(5,3,1) = a2_531 and RAO_Phase{2}(5,3,1) = p2_531.<p>
      | <b>Copyright (C) NTNU 2005</b></p>
      | <p><b>Author:</b> Oyvind N. Smogeli, 2005-05-03</p>
  "Waves " : $bdroot/Environment/Waves/Waves  spectrum_type=ITTC  disp_flag=on  plot_spectrum=off  plot_realization=off  hs=0.8  omega_peak=0  psi_mean=0  gamma=-1  spread=2  depth=inf  nfreq=20  ndir=10  energylim=0.005  freq_cutoff=3  dir_cutoff=0  rand_seed=123  rand_freq=on  rand_dir=on  Zeta_a=0  Omega=0  Phase=0  Wavenum=0  Psi=0
  zero-speed viiscous roll damping : Subsystem  mask{ABC=vesselABC}
      mask prompts: ABC "MSS vessel structure"
